simulink model "CT_PD_robot_2R"  (R2024a)
settings: Solver=ode4  StartTime=0.0  StopTime=6  FixedStep=0.001  RelTol=1e-3
model workspace (MAT data in the model file):
  p_hat.a1 = 1
  p_hat.a2 = 1
  p_hat.m1 = 2
  p_hat.m2 = 1
  p_hat.mm1 = 0.5
  p_hat.mm2 = 0.3
  p_hat.l1 = 0.5
  p_hat.l2 = 0.5
  p_hat.I1 = 0.166666666667
  p_hat.I2 = 0.0833333333333
  p_hat.kr1 = 50
  p_hat.kr2 = 50
  p_hat.Im1 = 0.0001
  p_hat.Im2 = 0.0001
  p_hat.g0 = 9.81
  p_real.a1 = 1
  p_real.a2 = 1
  p_real.m1 = 2
  p_real.m2 = 1
  p_real.mm1 = 0.5
  p_real.mm2 = 0.3
  p_real.l1 = 0.5
  p_real.l2 = 0.5
  p_real.I1 = 0.166666666667
  p_real.I2 = 0.0833333333333
  p_real.kr1 = 50
  p_real.kr2 = 50
  p_real.Im1 = 0.0001
  p_real.Im2 = 0.0001
  p_real.g0 = 9.81
undefined symbols (not defined in the file): d_amp, dq0, k_ct, k_dist, k_gp, k_noise, Kd, Kp, q0, seed, sig_dq, sig_q, t_d, Ts_n
settings Model: Creator=Mariapaola  LastModifiedBy=Mariapaola

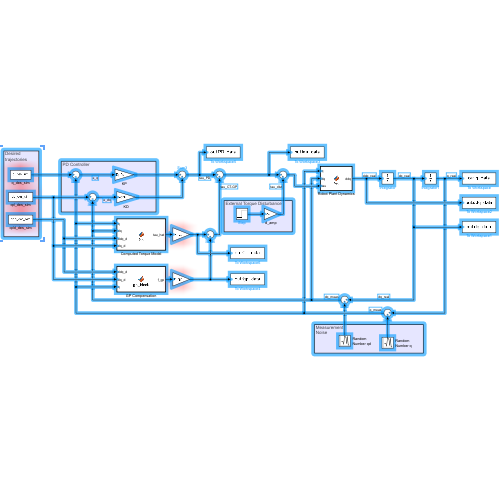
[thumbnail: Simulink's stored preview of the top-level diagram]
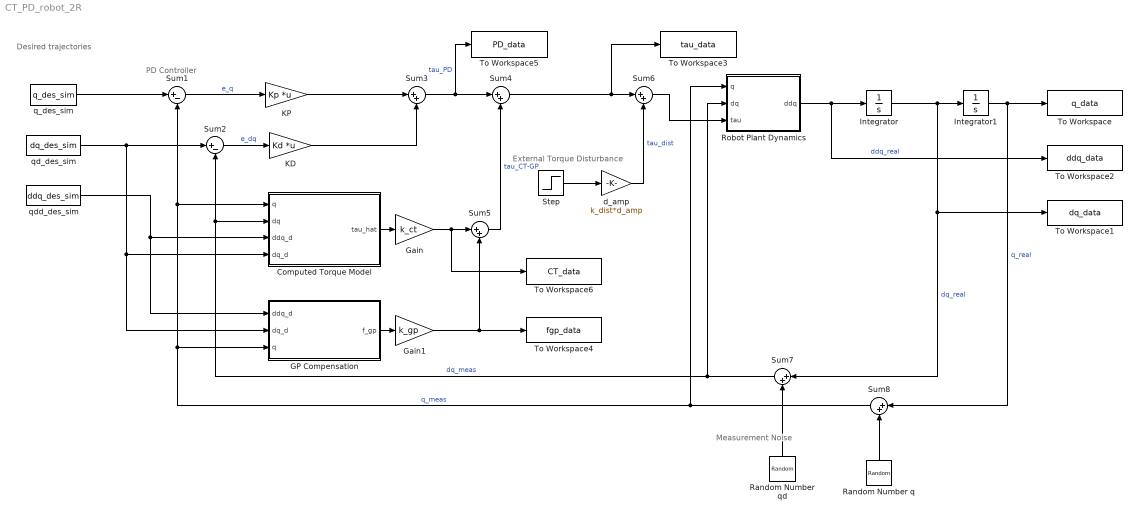
== system CT_PD_robot_2R ==
  note: Desired
      | trajectories
  note: PD Controller
  note: External Torque Disturbance
  note: Measurement
      | Noise
  Computed Torque Model : MATLAB Function  TreatAsAtomicUnit=on
  GP Compensation : MATLAB Function  TreatAsAtomicUnit=on
  Gain : Gain  Gain=k_ct
  Gain1 : Gain  Gain=k_gp
  Integrator : Integrator  InitialCondition=dq0
  Integrator1 : Integrator  InitialCondition=q0
  KD : Gain  Gain=Kd  Multiplication=Matrix(K*u)
  KP : Gain  Gain=Kp  Multiplication=Matrix(K*u)
  Random Number q : RandomNumber  Variance=k_noise*sig_q^2  Seed=seed  SampleTime=Ts_n
  Random Number qd : RandomNumber  Variance=k_noise*sig_dq^2  Seed=seed+1  SampleTime=Ts_n
  Robot Plant Dynamics : MATLAB Function  TreatAsAtomicUnit=on
  Step : Step  Time=t_d  SampleTime=0
  Sum1 : Sum  Inputs=|+-
  Sum2 : Sum  Inputs=|+-
  Sum{3..8} (6 alike) : Sum  Inputs=|++
  To Workspace : ToWorkspace  VariableName=q_data  SampleTime=-1
  To Workspace1 : ToWorkspace  VariableName=dq_data  SampleTime=-1
  To Workspace2 : ToWorkspace  VariableName=ddq_data  SampleTime=-1
  To Workspace3 : ToWorkspace  VariableName=tau_data  SampleTime=-1
  To Workspace4 : ToWorkspace  VariableName=fgp_data  SampleTime=-1
  To Workspace5 : ToWorkspace  VariableName=PD_data  SampleTime=-1
  To Workspace6 : ToWorkspace  VariableName=CT_data  SampleTime=-1
  d_amp : Gain  Gain=k_dist*d_amp
  "q_des_sim " : FromWorkspace  VariableName=q_des_sim
  qd_des_sim : FromWorkspace  VariableName=dq_des_sim
  qdd_des_sim : FromWorkspace  VariableName=ddq_des_sim
  wires:
  Robot Plant Dynamics/1(ddq) -> To Workspace2/1, Integrator/1  "ddq_real"
  Integrator/1 -> Sum7/1, To Workspace1/1, Integrator1/1  "dq_real"
  Integrator1/1 -> To Workspace/1, Sum8/1  "q_real"
  qdd_des_sim/1 -> GP Compensation/1(ddq_d), Computed Torque Model/3(ddq_d)
  Sum2/1 -> KD/1  "e_dq"
  Sum1/1 -> KP/1  "e_q"
  KP/1 -> Sum3/1
  KD/1 -> Sum3/2
  "q_des_sim "/1 -> Sum1/1
  qd_des_sim/1 -> GP Compensation/2(dq_d), Computed Torque Model/4(dq_d), Sum2/1
  Sum3/1 -> Sum4/1, To Workspace5/1  "tau_PD"
  GP Compensation/1(f_gp) -> Gain1/1
  Sum5/1 -> Sum4/2  "tau_CT-GP"
  Computed Torque Model/1(tau_hat) -> Gain/1
  Gain/1 -> To Workspace6/1, Sum5/1
  Gain1/1 -> Sum5/2, To Workspace4/1
  Sum4/1 -> Sum6/1, To Workspace3/1
  Sum6/1 -> Robot Plant Dynamics/3(tau)
  Step/1 -> d_amp/1
  d_amp/1 -> Sum6/2  "tau_dist"
  Sum7/1 -> Computed Torque Model/2(dq), Sum2/2, Robot Plant Dynamics/2(dq)  "dq_meas"
  Sum8/1 -> Robot Plant Dynamics/1(q), GP Compensation/3(q), Computed Torque Model/1(q), Sum1/2  "q_meas"
  Random Number q/1 -> Sum8/2
  Random Number qd/1 -> Sum7/2

== matlab function CT_PD_robot_2R/Computed Torque Model ==
  data: q input; tau_hat output; dq input; ddq_d input; dq_d input
function tau_hat = fcn(q,dq,ddq_d,dq_d)

tau_hat = computed_torque_model(q,dq,ddq_d,dq_d);

end

== matlab function CT_PD_robot_2R/Robot Plant Dynamics ==
  data: q input; ddq output; dq input; tau input
function ddq = fcn(q,dq,tau)

ddq = dynamics_model(q,dq,tau);

end

== matlab function CT_PD_robot_2R/GP Compensation ==
  data: ddq_d input; f_gp output; dq_d input; q input
function f_gp = gp_block(ddq_d, dq_d, q)
%#codegen
P = coder.load('gp_params.mat');
f_gp = gp_mean([ddq_d(:); dq_d(:); q(:)], P);
end
